simulink model "Simulink_DC_MG_4DGs_4Lines"  (R2024a)
settings: Solver=VariableStepAuto  StartTime=0.0  StopTime=10  RelTol=1e-3
InitFcn:
  | % In your simulation loop or callback function
  | for l = 1:numOfLines
  |     % Generate resistance disturbance (10% variation)
  |     delta_R_l = 0.1 * randn() * Line{l}.R;
  | 
  |     % Update the line resistance with disturbance
  |     Line{l}.R_disturbed = Line{l}.R + delta_R_l;
  | 
  |     % Use this disturbed value in your simulation equations
  |     % L_l * dI_l/dt = -Line{l}.R_disturbed * I_l + (V_i - V_j)
  | end
values from neighbouring files (symbols this model uses):
  Is = value(Is)    [implementTheorem1.m]    (also in implementTheorem1_Obj.m; implementTheorem1_debug.m = []; implementTheorem1_minLoss.m)
  K = sdpvar(1, 3, 'full')    [ComputePassivityForDGs.m]
  l = lines(k, 2)    [generatePhysicalTopology.m]    (also in ploting.m = legend({'\bf With Disturbance'},     'Location','southeast',)
  numOfDGs = size(B_il,1)    [centralizedLocalControlDesign.m]    (also in generateCommunicationTopology.m = size(coords, 1); globalControlDesign.m = size(B_il, 1); verifyControlConditions.m)
undefined symbols (not defined in the file or in its folder): Current_Load_activation, current_variance, D_Activation, DC_Activation, DG, LC_Activation, Line, line_variance, PlugIn, PlugOut, SS_Activation, V_nom, V_ref, voltage_variance
libraries: spsSeriesRLCBranchLib x28, spsControlledCurrentSourceLib x12, spsCurrentMeasurementLib x8, simulink x4, spsIdealSwitchLib x4, spsStairGeneratorLib x4, spsControlledVoltageSourceLib x4, spsDCVoltageSourceLib x4, spsDiodeLib x4, spsIGBTLib x4, spsVoltageMeasurementLib x4, spspowerguiLib x1
(part 2 of 2)

== system Simulink_DC_MG_4DGs_4Lines/Subsystem6/Disturbance activation1 ==
  Clock : Clock
  Constant1 : Constant  Value=D_Activation
  Relational Operator : RelationalOperator  OutDataTypeStr=boolean  RndMeth=Simplest  InputSameDT=off
  Out1 : Outport  VectorParamsAs1DForOutWhenUnconnected=off
  wires:
  Clock/1 -> Relational Operator/1
  Relational Operator/1 -> Out1/1
  Constant1/1 -> Relational Operator/2

== system Simulink_DC_MG_4DGs_4Lines/Transmission Line 1/Disturbance activation ==
  Clock : Clock
  Constant1 : Constant  Value=D_Activation
  Relational Operator : RelationalOperator  OutDataTypeStr=boolean  RndMeth=Simplest  InputSameDT=off
  Out1 : Outport  VectorParamsAs1DForOutWhenUnconnected=off
  wires:
  Clock/1 -> Relational Operator/1
  Relational Operator/1 -> Out1/1
  Constant1/1 -> Relational Operator/2

== system Simulink_DC_MG_4DGs_4Lines/Transmission Line 2/Disturbance activation ==
  Clock : Clock
  Constant1 : Constant  Value=D_Activation
  Relational Operator : RelationalOperator  OutDataTypeStr=boolean  RndMeth=Simplest  InputSameDT=off
  Out1 : Outport  VectorParamsAs1DForOutWhenUnconnected=off
  wires:
  Clock/1 -> Relational Operator/1
  Relational Operator/1 -> Out1/1
  Constant1/1 -> Relational Operator/2

== system Simulink_DC_MG_4DGs_4Lines/Transmission Line 3/Disturbance activation ==
  Clock : Clock
  Constant1 : Constant  Value=D_Activation
  Relational Operator : RelationalOperator  OutDataTypeStr=boolean  RndMeth=Simplest  InputSameDT=off
  Out1 : Outport  VectorParamsAs1DForOutWhenUnconnected=off
  wires:
  Clock/1 -> Relational Operator/1
  Relational Operator/1 -> Out1/1
  Constant1/1 -> Relational Operator/2

== system Simulink_DC_MG_4DGs_4Lines/Transmission Line4/Disturbance activation ==
  Clock : Clock
  Constant1 : Constant  Value=D_Activation
  Relational Operator : RelationalOperator  OutDataTypeStr=boolean  RndMeth=Simplest  InputSameDT=off
  Out1 : Outport  VectorParamsAs1DForOutWhenUnconnected=off
  wires:
  Clock/1 -> Relational Operator/1
  Relational Operator/1 -> Out1/1
  Constant1/1 -> Relational Operator/2

== system Simulink_DC_MG_4DGs_4Lines/Local and Global Controller /Subsystem/Distributed Controller Activation ==
  Clock : Clock
  Constant1 : Constant  Value=DC_Activation
  Relational Operator : RelationalOperator  OutDataTypeStr=boolean  RndMeth=Simplest  InputSameDT=off
  Out1 : Outport  VectorParamsAs1DForOutWhenUnconnected=off
  wires:
  Constant1/1 -> Relational Operator/2
  Relational Operator/1 -> Out1/1
  Clock/1 -> Relational Operator/1

== system Simulink_DC_MG_4DGs_4Lines/Local and Global Controller /Subsystem/Local Controller Activation ==
  Clock : Clock
  Constant1 : Constant  Value=LC_Activation
  Relational Operator : RelationalOperator  OutDataTypeStr=boolean  RndMeth=Simplest  InputSameDT=off
  Out1 : Outport  VectorParamsAs1DForOutWhenUnconnected=off
  wires:
  Relational Operator/1 -> Out1/1
  Constant1/1 -> Relational Operator/2
  Clock/1 -> Relational Operator/1

== system Simulink_DC_MG_4DGs_4Lines/Local and Global Controller /Subsystem/Steady State Control Activation ==
  Clock : Clock
  Constant1 : Constant  Value=SS_Activation
  Relational Operator : RelationalOperator  OutDataTypeStr=boolean  RndMeth=Simplest  InputSameDT=off
  Out1 : Outport  VectorParamsAs1DForOutWhenUnconnected=off
  wires:
  Clock/1 -> Relational Operator/1
  Relational Operator/1 -> Out1/1
  Constant1/1 -> Relational Operator/2

== system Simulink_DC_MG_4DGs_4Lines/Local and Global Controller /Subsystem/Subsystem2 ==
  u : Inport
  0.05 : Gain
  Relational Operator : RelationalOperator  OutDataTypeStr=boolean  InputSameDT=off
  Scope : Scope  NumInputPorts=2
  Scope2 : Scope
  Triangle1 : simulink/Sources/Repeating Sequence  rep_seq_t=[0 40e-5 80e-5]  rep_seq_y=[0 1 0]
  PWM : Outport
  wires:
  0.05/1 -> Relational Operator/1, Scope/1
  Triangle1/1 -> Relational Operator/2, Scope/2
  u/1 -> 0.05/1
  Relational Operator/1 -> PWM/1, Scope2/1

== system Simulink_DC_MG_4DGs_4Lines/Local and Global Controller /Subsystem1/Distributed Controller Activation ==
  Clock : Clock
  Constant1 : Constant  Value=DC_Activation
  Relational Operator : RelationalOperator  OutDataTypeStr=boolean  RndMeth=Simplest  InputSameDT=off
  Out1 : Outport  VectorParamsAs1DForOutWhenUnconnected=off
  wires:
  Constant1/1 -> Relational Operator/2
  Relational Operator/1 -> Out1/1
  Clock/1 -> Relational Operator/1

== system Simulink_DC_MG_4DGs_4Lines/Local and Global Controller /Subsystem1/Local Controller Activation ==
  Clock : Clock
  Constant1 : Constant  Value=LC_Activation
  Relational Operator : RelationalOperator  OutDataTypeStr=boolean  RndMeth=Simplest  InputSameDT=off
  Out1 : Outport  VectorParamsAs1DForOutWhenUnconnected=off
  wires:
  Relational Operator/1 -> Out1/1
  Constant1/1 -> Relational Operator/2
  Clock/1 -> Relational Operator/1

== system Simulink_DC_MG_4DGs_4Lines/Local and Global Controller /Subsystem1/Steady State Control Activation ==
  Clock : Clock
  Constant1 : Constant  Value=SS_Activation
  Relational Operator : RelationalOperator  OutDataTypeStr=boolean  RndMeth=Simplest  InputSameDT=off
  Out1 : Outport  VectorParamsAs1DForOutWhenUnconnected=off
  wires:
  Clock/1 -> Relational Operator/1
  Relational Operator/1 -> Out1/1
  Constant1/1 -> Relational Operator/2

== system Simulink_DC_MG_4DGs_4Lines/Local and Global Controller /Subsystem1/Subsystem2 ==
  u : Inport
  0.05 : Gain
  Relational Operator : RelationalOperator  OutDataTypeStr=boolean  InputSameDT=off
  Scope : Scope  NumInputPorts=2
  Scope2 : Scope
  Triangle1 : simulink/Sources/Repeating Sequence  rep_seq_t=[0 40e-5 80e-5]  rep_seq_y=[0 1 0]
  PWM : Outport
  wires:
  0.05/1 -> Relational Operator/1, Scope/1
  Triangle1/1 -> Relational Operator/2, Scope/2
  u/1 -> 0.05/1
  Relational Operator/1 -> PWM/1, Scope2/1

== system Simulink_DC_MG_4DGs_4Lines/Local and Global Controller /Subsystem2/Distributed Controller Activation ==
  Clock : Clock
  Constant1 : Constant  Value=DC_Activation
  Relational Operator : RelationalOperator  OutDataTypeStr=boolean  RndMeth=Simplest  InputSameDT=off
  Out1 : Outport  VectorParamsAs1DForOutWhenUnconnected=off
  wires:
  Constant1/1 -> Relational Operator/2
  Relational Operator/1 -> Out1/1
  Clock/1 -> Relational Operator/1

== system Simulink_DC_MG_4DGs_4Lines/Local and Global Controller /Subsystem2/Local Controller Activation ==
  Clock : Clock
  Constant1 : Constant  Value=LC_Activation
  Relational Operator : RelationalOperator  OutDataTypeStr=boolean  RndMeth=Simplest  InputSameDT=off
  Out1 : Outport  VectorParamsAs1DForOutWhenUnconnected=off
  wires:
  Relational Operator/1 -> Out1/1
  Constant1/1 -> Relational Operator/2
  Clock/1 -> Relational Operator/1

== system Simulink_DC_MG_4DGs_4Lines/Local and Global Controller /Subsystem2/Steady State Control Activation ==
  Clock : Clock
  Constant1 : Constant  Value=SS_Activation
  Relational Operator : RelationalOperator  OutDataTypeStr=boolean  RndMeth=Simplest  InputSameDT=off
  Out1 : Outport  VectorParamsAs1DForOutWhenUnconnected=off
  wires:
  Clock/1 -> Relational Operator/1
  Relational Operator/1 -> Out1/1
  Constant1/1 -> Relational Operator/2

== system Simulink_DC_MG_4DGs_4Lines/Local and Global Controller /Subsystem2/Subsystem2 ==
  u : Inport
  0.05 : Gain
  Relational Operator : RelationalOperator  OutDataTypeStr=boolean  InputSameDT=off
  Scope : Scope  NumInputPorts=2
  Scope2 : Scope
  Triangle1 : simulink/Sources/Repeating Sequence  rep_seq_t=[0 40e-5 80e-5]  rep_seq_y=[0 1 0]
  PWM : Outport
  wires:
  0.05/1 -> Relational Operator/1, Scope/1
  Triangle1/1 -> Relational Operator/2, Scope/2
  u/1 -> 0.05/1
  Relational Operator/1 -> PWM/1, Scope2/1

== system Simulink_DC_MG_4DGs_4Lines/Local and Global Controller /Subsystem3/Distributed Controller Activation ==
  Clock : Clock
  Constant1 : Constant  Value=DC_Activation
  Relational Operator : RelationalOperator  OutDataTypeStr=boolean  RndMeth=Simplest  InputSameDT=off
  Out1 : Outport  VectorParamsAs1DForOutWhenUnconnected=off
  wires:
  Constant1/1 -> Relational Operator/2
  Relational Operator/1 -> Out1/1
  Clock/1 -> Relational Operator/1

== system Simulink_DC_MG_4DGs_4Lines/Local and Global Controller /Subsystem3/Local Controller Activation ==
  Clock : Clock
  Constant1 : Constant  Value=LC_Activation
  Relational Operator : RelationalOperator  OutDataTypeStr=boolean  RndMeth=Simplest  InputSameDT=off
  Out1 : Outport  VectorParamsAs1DForOutWhenUnconnected=off
  wires:
  Relational Operator/1 -> Out1/1
  Constant1/1 -> Relational Operator/2
  Clock/1 -> Relational Operator/1

== system Simulink_DC_MG_4DGs_4Lines/Local and Global Controller /Subsystem3/Steady State Control Activation ==
  Clock : Clock
  Constant1 : Constant  Value=SS_Activation
  Relational Operator : RelationalOperator  OutDataTypeStr=boolean  RndMeth=Simplest  InputSameDT=off
  Out1 : Outport  VectorParamsAs1DForOutWhenUnconnected=off
  wires:
  Clock/1 -> Relational Operator/1
  Relational Operator/1 -> Out1/1
  Constant1/1 -> Relational Operator/2

== system Simulink_DC_MG_4DGs_4Lines/Local and Global Controller /Subsystem3/Subsystem2 ==
  u : Inport
  0.05 : Gain
  Relational Operator : RelationalOperator  OutDataTypeStr=boolean  InputSameDT=off
  Scope : Scope  NumInputPorts=2
  Scope2 : Scope
  Triangle1 : simulink/Sources/Repeating Sequence  rep_seq_t=[0 40e-5 80e-5]  rep_seq_y=[0 1 0]
  PWM : Outport
  wires:
  0.05/1 -> Relational Operator/1, Scope/1
  Triangle1/1 -> Relational Operator/2, Scope/2
  u/1 -> 0.05/1
  Relational Operator/1 -> PWM/1, Scope2/1
